simulink model "mcpherson_scaling"  (R2025b)
settings: Solver=VariableStepAuto  StartTime=0.0  StopTime=1e3  RelTol=1e-3  AbsTol=1e-3
libraries: customization_lib x11, fl_lib x3, nesl_utility x2
settings Model: Creator=degoede  LastModifiedBy=ndegoede
settings SolverCC: AutoScaleAbsTol=off
settings SimscapeCC: SimscapeLogType=all  SimscapeLogSimulationStatistics=on  SimscapeLogOpenViewer=on

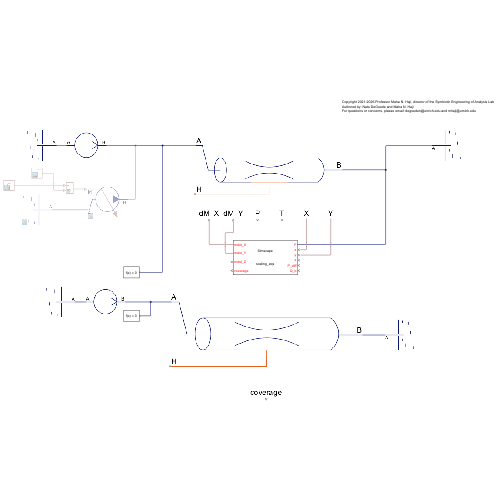
[thumbnail: Simulink's stored preview of the top-level diagram]
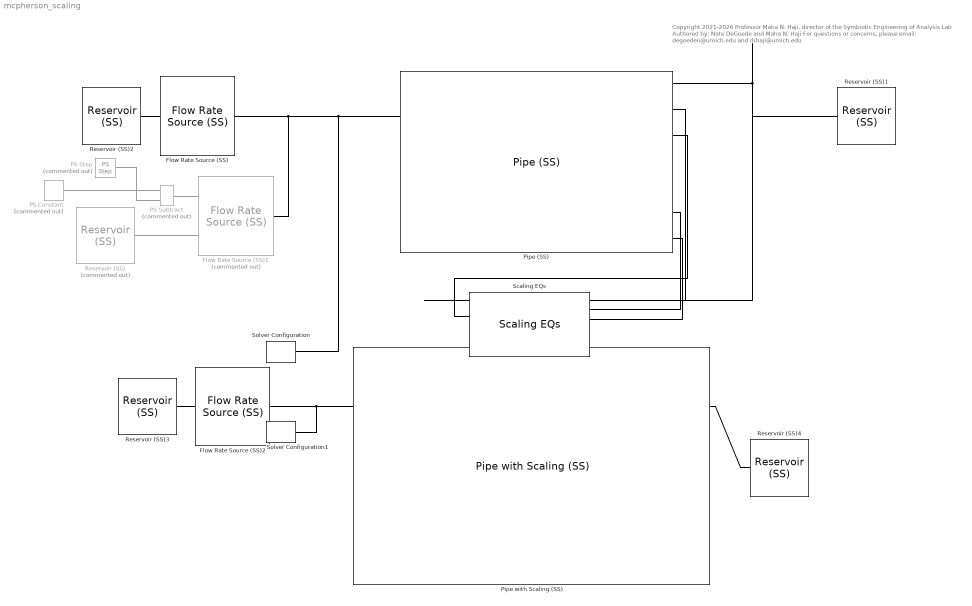
== system mcpherson_scaling ==
  note: Copyright 2021-2026 Professor Maha N. Haji, director of the Symbiotic Engineering of Analysis Lab
      | Authored by: Nate DeGoede and Maha N. Haji
      | For questions or concerns, please email: degoeden@umich.edu and mhaji@umich.edu
  Flow Rate Source (SS) : customization_lib/solution/sources/Flow Rate Source (SS)  source_type=foundation.enum.constant_controlled.constant  flow_type=foundation.enum.mass_volumetric_flow.volumetric  mass_flow=0 kg/s  volumetric_flow=2e-3 lpm  power_spec=foundation.enum.power_spec.isentropic  area=0.1 m^2  custom_ports=false  length_A=1e-3 m  length_B=1e-3 m
      settings: SourceProductName=Customization  InternalSimscapePortConfiguration="{\"Bottom\":[],\"Left\":[{\"id\":\"A\",\"label\":\"A\",\"type\":\"customization.solution.solution\"}],\"Right\":[{\"id\":\"B\",\"label\":\"B\",\"type\":\"customization.solution.solution\"}],\"Top\":[]}"
  Flow Rate Source (SS)1 : customization_lib/solution/sources/Flow Rate Source (SS)  Commented=on  source_type=foundation.enum.constant_controlled.controlled  flow_type=foundation.enum.mass_volumetric_flow.mass  mass_flow=0 kg/s  volumetric_flow=0.001 m^3/s  power_spec=foundation.enum.power_spec.isentropic  area=0.1 m^2  custom_ports=false  length_A=1e-3 m  length_B=1e-3 m
      settings: SourceProductName=Customization  InternalSimscapePortConfiguration="{\"Bottom\":[],\"Left\":[{\"id\":\"A\",\"label\":\"A\",\"type\":\"customization.solution.solution\"},{\"id\":\"M\",\"label\":\"M\",\"type\":\"input\"}],\"Right\":[{\"id\":\"B\",\"label\":\"B\",\"type\":\"customization.solution.solution\"}],\"Top\":[]}"
  Flow Rate Source (SS)2 : customization_lib/solution/sources/Flow Rate Source (SS)  source_type=foundation.enum.constant_controlled.constant  flow_type=foundation.enum.mass_volumetric_flow.volumetric  mass_flow=0 kg/s  volumetric_flow=2e-3 lpm  power_spec=foundation.enum.power_spec.isentropic  area=0.1 m^2  custom_ports=false  length_A=1e-3 m  length_B=1e-3 m
      settings: SourceProductName=Customization  InternalSimscapePortConfiguration="{\"Bottom\":[],\"Left\":[{\"id\":\"A\",\"label\":\"A\",\"type\":\"customization.solution.solution\"}],\"Right\":[{\"id\":\"B\",\"label\":\"B\",\"type\":\"customization.solution.solution\"}],\"Top\":[]}"
  PS Constant : fl_lib/Physical Signals/Sources/PS Constant  Commented=on  constant=0.1 kg/s
  PS Step : fl_lib/Physical Signals/Sources/PS Step  Commented=on  step_time=5e2 s  initial_value=0.1 kg/s  final_value=0 kg/s
  PS Subtract : fl_lib/Physical Signals/Functions/PS Subtract  Commented=on
  Pipe (SS) : customization_lib/solution/elements/Pipe (SS)  length=1 cm  area=1 cm^2  Dh=2*(1^0.5)/pi cm  Re_min=0.1  length_add=0 m  roughness=1.5e-05 m  Re_lam=2000  Re_tur=4000  shape_factor=64  Nu_lam=3.66  dynamic_compressibility=true  dM_X_source=true  dM_Y_source=true  dM_Z_source=false  dM_W_source=false  phi_source=false  inertia=false  p0=1 atm  T0=293.15 K  x0=55.4 kg/m^3  y0=0 kg/m^3  z0=0 kg/m^3  mdot0=0 kg/s  m_measure=false  p_measure=true  t_measure=true  pi_measure=false  x_measure=true  y_measure=true  z_measure=false  internal_concentration_gradient=false  flux_area=7.4 m^2  custom_ports=false  length_A=1e-3 m  length_B=1e-3 m
      settings: SourceProductName=Customization  InternalSimscapePortConfiguration="{\"Bottom\":[{\"id\":\"dM_X\",\"label\":\"dM_X\",\"type\":\"input\"},{\"id\":\"dM_Y\",\"label\":\"dM_Y\",\"type\":\"input\"},{\"id\":\"P\",\"label\":\"P\",\"type\":\"output\"},{\"id\":\"T\",\"label\":\"T\",\"type\":\"output\"},{\"id\":\"X\",\"label\":\"X\",\"type\":\"output\"},{\"id\":\"Y\",\"label\":\"Y\",\"type\":\"output\"}],\"Left\":[{\"id\":\"A\",\"label\":\"A\",\"type\":\"customization.solution.solution\"},{\"id\":\"H\",\"label\":\"H\",\"type\":\"foundation.thermal.thermal\"}],\"Right\":[{\"id\":\"B\",\"label\":\"B\",\"type\":\"customization.solution.solution\"}],\"Top\":[]}"
  Pipe with Scaling (SS) : customization_lib/scaling/Pipe with Scaling (SS)  length=1 cm  area=1 cm^2  Dh=2*(1^0.5)/pi cm  perimeter=0.1 cm  Re_min=0.1  length_add=1 m  roughness=15e-6 m  Re_lam=2000  Re_tur=4000  shape_factor=64  Nu_lam=3.66  dynamic_compressibility=true  dM_X_source=false  dM_Y_source=false  dM_Z_source=false  dM_W_source=false  phi_source=false  inertia=false  p0=1 atm  T0=293.15 K  x0=55.4 kg/m^3  y0=0 kg/m^3  z0=0 kg/m^3  mdot0=0 kg/s  m_measure=false  p_measure=false  t_measure=false  pi_measure=false  x_measure=false  y_measure=false  z_measure=false  internal_concentration_gradient=false  flux_area=7.4 m^2  custom_ports=false  length_A=1e-3 m  length_B=1e-3 m  scaling_x=true  x_eq=5.89e-3 g/l  K_G_x=6.0463e-7 m/s  s_x=1  A_nucleation_x=6.6329e-13 m^2  aspect_ratio_x=0.9163  scales_per_area_x=3e4 1/cm^2  alpha_x=1000 1/m  F_detach_x=1e3 N  F_detach_buffer_x=1e-3 N  Mscale_x0=0 kg  scaling_y=false  y_eq=1e15 g/l  K_G_y=0 m/s  s_y=1  A_nucleation_y=1e-30 m^2  aspect_ratio_y=0.9  scales_per_area_y=0 1/cm^2  alpha_y=1000 1/m  F_detach_y=1 N  F_detach_buffer_y=1e-3 N  Mscale_y0=0 kg  scaling_z=false  z_eq=1e15 g/l  K_G_z=0 m/s  s_z=1  A_nucleation_z=1e-30 m^2  aspect_ratio_z=0.9  scales_per_area_z=0 1/cm^2  alpha_z=1000 1/m  F_detach_z=1 Pa  F_detach_buffer_z=1e-3 N  Mscale_z0=0 kg
      settings: SourceProductName=Customization  InternalSimscapePortConfiguration="{\"Bottom\":[{\"id\":\"coverage\",\"label\":\"coverage\",\"type\":\"output\"}],\"Left\":[{\"id\":\"A\",\"label\":\"A\",\"type\":\"customization.solution.solution\"},{\"id\":\"H\",\"label\":\"H\",\"type\":\"foundation.thermal.thermal\"}],\"Right\":[{\"id\":\"B\",\"label\":\"B\",\"type\":\"customization.solution.solution\"}],\"Top\":[]}"
  Reservoir (SS) : customization_lib/solution/elements/Reservoir (SS)  Commented=on  pressure_spec=foundation.enum.pressure_spec.atmospheric  reservoir_pressure=1 atm  reservoir_temperature=293.15 K  reservoir_concentration=0 kg/m^3  reservoir_concentration_y=0 kg/m^3  reservoir_concentration_z=0 kg/m^3  area=1 cm^2  custom_ports=false  length_A=1e-3 m
      settings: SourceProductName=Customization  InternalSimscapePortConfiguration="{\"Bottom\":[],\"Left\":[{\"id\":\"A\",\"label\":\"A\",\"type\":\"customization.solution.solution\"}],\"Right\":[],\"Top\":[]}"
  Reservoir (SS)1 : customization_lib/solution/elements/Reservoir (SS)  pressure_spec=foundation.enum.pressure_spec.atmospheric  reservoir_pressure=0.101325 MPa  reservoir_temperature=293.15 K  reservoir_concentration=0 kg/m^3  reservoir_concentration_y=0 kg/m^3  reservoir_concentration_z=0 kg/m^3  area=27 mm^2  custom_ports=false  length_A=1e-3 m
      settings: SourceProductName=Customization  InternalSimscapePortConfiguration="{\"Bottom\":[],\"Left\":[{\"id\":\"A\",\"label\":\"A\",\"type\":\"customization.solution.solution\"}],\"Right\":[],\"Top\":[]}"
  Reservoir (SS)2 : customization_lib/solution/elements/Reservoir (SS)  pressure_spec=foundation.enum.pressure_spec.atmospheric  reservoir_pressure=2 atm  reservoir_temperature=293.15 K  reservoir_concentration=55.4 kg/m^3  reservoir_concentration_y=0 kg/m^3  reservoir_concentration_z=0 kg/m^3  area=1 cm^2  custom_ports=false  length_A=1e-3 m
      settings: SourceProductName=Customization  InternalSimscapePortConfiguration="{\"Bottom\":[],\"Left\":[{\"id\":\"A\",\"label\":\"A\",\"type\":\"customization.solution.solution\"}],\"Right\":[],\"Top\":[]}"
  Reservoir (SS)3 : customization_lib/solution/elements/Reservoir (SS)  pressure_spec=foundation.enum.pressure_spec.atmospheric  reservoir_pressure=2 atm  reservoir_temperature=293.15 K  reservoir_concentration=55.4 kg/m^3  reservoir_concentration_y=0 kg/m^3  reservoir_concentration_z=0 kg/m^3  area=1 cm^2  custom_ports=false  length_A=1e-3 m
      settings: SourceProductName=Customization  InternalSimscapePortConfiguration="{\"Bottom\":[],\"Left\":[{\"id\":\"A\",\"label\":\"A\",\"type\":\"customization.solution.solution\"}],\"Right\":[],\"Top\":[]}"
  Reservoir (SS)4 : customization_lib/solution/elements/Reservoir (SS)  pressure_spec=foundation.enum.pressure_spec.atmospheric  reservoir_pressure=0.101325 MPa  reservoir_temperature=293.15 K  reservoir_concentration=0 kg/m^3  reservoir_concentration_y=0 kg/m^3  reservoir_concentration_z=0 kg/m^3  area=27 mm^2  custom_ports=false  length_A=1e-3 m
      settings: SourceProductName=Customization  InternalSimscapePortConfiguration="{\"Bottom\":[],\"Left\":[{\"id\":\"A\",\"label\":\"A\",\"type\":\"customization.solution.solution\"}],\"Right\":[],\"Top\":[]}"
  Scaling EQs : customization_lib/scaling/Scaling EQs  scaling_x=true  scaling_y=false  scaling_z=false  A_max=0.1 cm^2  x_eq=5.89e-3 kg/m^3  K_G=6.0463e-7 m/s  s=1  A_nucleation=6.6329e-13 m^2  aspect_ratio=0.9163  scales_per_area=3e4 1/cm^2  F_detach=1e3 N  alpha=1000 1/m  F_detach_buffer=1e-3 N  y_eq=1000 kg/m^3  K_G_y=1e-30 m/s  s_y=1  A_nucleation_y=1e-30 m^2  aspect_ratio_y=0.9  scales_per_area_y=1 1/m^2  F_detach_y=1 N  alpha_y=1000 1/m  F_detach_buffer_y=1e-3 N  z_eq=1 kg/m^3  K_G_z=1 m/s  s_z=1  A_nucleation_z=1e-5 m^2  aspect_ratio_z=1  scales_per_area_z=1 1/m^2  F_detach_z=1 Pa  alpha_z=1000 1/m  F_detach_buffer_z=1e-3 N  Mscale_x0=0 kg  Mscale_y0=0 kg  Mscale_z0=0 kg
      settings: SourceProductName=Customization  InternalSimscapePortConfiguration="{\"Bottom\":[],\"Left\":[{\"id\":\"F\",\"label\":\"F\",\"type\":\"customization.solution.solution\"},{\"id\":\"x\",\"label\":\"x\",\"type\":\"input\"},{\"id\":\"y\",\"label\":\"y\",\"type\":\"input\"},{\"id\":\"z\",\"label\":\"z\",\"type\":\"input\"},{\"id\":\"P_diff\",\"label\":\"P_diff\",\"type\":\"input\"},{\"id\":\"Q_b\",\"label\":\"Q_b\",\"type\":\"input\"}],\"Right\":[{\"id\":\"mdot_x\",\"label\":\"mdot_X\",\"type\":\"output\"},{\"id\":\"mdot_y\",\"label\":\"mdot_Y\",\"type\":\"output\"},{\"id\":\"mdot_z\",\"label\":\"mdot_Z\",\"type\":\"output\"},{\"id\":\"coverage\",\"label\":\"coverage\",\"type\":\"output\"}],\"Top\":[]}"
  Solver Configuration : nesl_utility/Solver Configuration  PhysicalDomain=network_engine_domain  SubClassName=solver  LeftPortType=input  RightPortType=generic  Tones=[]  Harmonics=[]  SimulateNoise=off  Profile=off  UseLocalSampling=off  EnableSwitchedLinearOptims=on  FrequencyDomain=off  UseCCode=off  RelTol=0.001  AbsTol=0.001  MinStep=1e-09  ToWorkspace=off  RevertToSquareIcSolve=off  NumHomotopyIterations=100  PhasorMode=off  PhasorModeNumHarmonics=1  ConsistencySolver=NEWTON_XTOL_AFTER_FTOL  IndexReductionMethod=DerivativeReplacement  DoDC=off  ResidualTolerance=1e-09  ConsistencyTolSource=GLOBAL  ConsistencyAbsTol=0.001  ConsistencyRelTol=0.001  ConsistencyTolFactor=0.001  UseLocalSolver=off  LocalSolverChoice=NE_BACKWARD_EULER_ADVANCER  ResolveIndetEquations=on  FunctionEvalNumThread=1  LocalSolverSampleTime=0.001  DoFixedCost=off  MaxNonlinIter=3  MaxModeIter=2  ComputeImpulses=off  ImpulseIterations=2  LinearAlgebra=auto  LinearAlgebraNumThread=0  EquationFormulation=NE_TIME_EF  DelaysMemoryBudget=1024  AutomaticFiltering=off  FilteringTimeConstant=0.001  PartitionStorageMethod=AS_NEEDED  PartitionMemoryBudget=1024  PartitionMethod=ROBUST  MultibodyUseLocalSolver=off  MultibodyLocalSolverChoice=ODE1  MultibodyLocalSolverSampleTime=0.001
  Solver Configuration1 : nesl_utility/Solver Configuration  PhysicalDomain=network_engine_domain  SubClassName=solver  LeftPortType=input  RightPortType=generic  Tones=[]  Harmonics=[]  SimulateNoise=off  Profile=off  UseLocalSampling=off  EnableSwitchedLinearOptims=on  FrequencyDomain=off  UseCCode=off  RelTol=0.001  AbsTol=0.001  MinStep=1e-09  ToWorkspace=off  RevertToSquareIcSolve=off  NumHomotopyIterations=100  PhasorMode=off  PhasorModeNumHarmonics=1  ConsistencySolver=NEWTON_XTOL_AFTER_FTOL  IndexReductionMethod=DerivativeReplacement  DoDC=off  ResidualTolerance=1e-09  ConsistencyTolSource=GLOBAL  ConsistencyAbsTol=0.001  ConsistencyRelTol=0.001  ConsistencyTolFactor=0.001  UseLocalSolver=off  LocalSolverChoice=NE_BACKWARD_EULER_ADVANCER  ResolveIndetEquations=on  FunctionEvalNumThread=1  LocalSolverSampleTime=0.001  DoFixedCost=off  MaxNonlinIter=3  MaxModeIter=2  ComputeImpulses=off  ImpulseIterations=2  LinearAlgebra=auto  LinearAlgebraNumThread=0  EquationFormulation=NE_TIME_EF  DelaysMemoryBudget=1024  AutomaticFiltering=off  FilteringTimeConstant=0.001  PartitionStorageMethod=AS_NEEDED  PartitionMemoryBudget=1024  PartitionMethod=ROBUST  MultibodyUseLocalSolver=off  MultibodyLocalSolverChoice=ODE1  MultibodyLocalSolverSampleTime=0.001
  connections:
  Pipe (SS)/LConn1 -- Solver Configuration/RConn1 -- Flow Rate Source (SS)1/RConn1 -- Flow Rate Source (SS)/RConn1
  Pipe (SS)/RConn1 -- Reservoir (SS)1/LConn1 -- Scaling EQs/LConn1
  Scaling EQs/LConn2 -- Pipe (SS)/RConn6
  Flow Rate Source (SS)/LConn1 -- Reservoir (SS)2/LConn1
  PS Step/RConn1 -- PS Subtract/LConn2
  PS Constant/RConn1 -- PS Subtract/LConn1
  PS Subtract/RConn1 -- Flow Rate Source (SS)1/LConn2
  Reservoir (SS)/LConn1 -- Flow Rate Source (SS)1/LConn1
  Scaling EQs/LConn3 -- Pipe (SS)/RConn7
  Flow Rate Source (SS)2/RConn1 -- Pipe with Scaling (SS)/LConn1 -- Solver Configuration1/RConn1
  Flow Rate Source (SS)2/LConn1 -- Reservoir (SS)3/LConn1
  Reservoir (SS)4/LConn1 -- Pipe with Scaling (SS)/RConn1
  Scaling EQs/RConn1 -- Pipe (SS)/RConn2
  Scaling EQs/RConn2 -- Pipe (SS)/RConn3
